simulink model "drone_position_control_ista_tuned"  (R2022a)
settings: Solver=ode4  StartTime=0.0  StopTime=42  FixedStep=.0005  RelTol=1e-3
model workspace (MAT data in the model file):
  AttDyna_Ixx = 0.0211
  AttDyna_Iyy = 0.0219
  AttDyna_Izz = 0.0366
  AttDyna_JRP = 0.0001287
  ConEfficiency_drone_R = 0.225
  ConEfficiency_drone_cM = 1.779e-07
  ConEfficiency_drone_cT = 1.105e-05
  HeightISTAParams = [20 40 0.01 -22 8 8 0.005 3 5]
  HeightNominalPlant = [1.4 9.8 1.105e-05 1148 -141.4]
  HeightSTAParams = [20 12 0.01 -22 8 8 0.005 3 5]
  PosDyna_GravityAcc = 9.8
  PosDyna_Mass = 1.4
  PowerUnit_CR = 1148
  PowerUnit_Tm = 0.02
  PowerUnit_wb = -141.4
  XYISTAParams = [3 1 0.005 -1.7 1.7 1.7 0.005 1.5]
undefined symbols (not defined in the file): earthRadius, Receive, Send
libraries: aerolibfltsims x3, slpidlib x3, aerolibanimutils x1
(part 2 of 2)

== matlab function drone_position_control_ista_tuned/水平和高度控制/ISTA_y_velocity/ISTA_formula ==
  data: e input; u output; nu input; parameters input; nu_next output; velocity input
function [u, nu_next] = ista_velocity_tuned(e, nu, parameters, velocity)
%#codegen
% 改进隐式ISTA：参数 [k1 k2 epsilon amin amax nu_max Ts lambda]。
% epsilon>0 使用边界层隐式解；epsilon=0 为原作者隐式核。
k1=parameters(1);k2=parameters(2);epsilon=parameters(3);
lo=parameters(4);hi=parameters(5);nu_max=parameters(6);
h=parameters(7);lambda=parameters(8);
if epsilon>0
 [u_ista,nu_candidate]=ista_compensated_step(e,nu,k1,k2,h,epsilon);
else
 [u_ista,nu_candidate]=ISTA_author_step(-e,nu,k1,k2,h,0);
end
u_raw=-lambda*velocity+u_ista;
u=min(max(u_raw,lo),hi);
dnu=nu_candidate-nu;
if (u_raw>hi&&dnu>0)||(u_raw<lo&&dnu<0)
 nu_candidate=nu;
end
nu_next=min(max(nu_candidate,-nu_max),nu_max);
end

function [u, nu_candidate, s_pred] = ista_compensated_step(s, nu, k1, k2, Ts, epsilon)
%#codegen
% 工程改进：用积分状态近似补偿未知加速度扰动，修正隐式预测。
% 假设局部误差动力学 s_dot=-u-d；nu在稳态提供-d的补偿。
% 因而采用 d_hat=-nu，预测 s_pred=s-Ts*(u-nu)。
% 与nu_next=nu+Ts*k2*sat(s_pred/epsilon)、u=k1*psi(s_pred)+nu_next联立。
% 把原核输入平移Ts*nu后，消元右端从s-Ts*nu变为s。
% 不读取实际扰动力；nu并不是任何瞬态下都准确的扰动观测器。
% 这是作者名义隐式核的工程扩展，不等同作者原函数。
[u,nu_candidate,s_pred]=ista_regularized_step(s+Ts*nu,nu,k1,k2,Ts,epsilon);
end

function [u, nu_candidate, s_pred] = ista_regularized_step(s, nu, k1, k2, Ts, epsilon)
%#codegen
% 边界层隐式 ISTA 工程扩展；不是作者原函数的原样复制。
% s = 目标速度 - 实际速度，nu 是当前积分状态，Ts 是控制采样周期。
% epsilon > 0 是速度误差边界层宽度，单位与 s 相同。
%
% 将下面三个名义、未限幅的离散方程联合求解：
% s_pred       = s - Ts*u
% nu_candidate = nu + Ts*k2*sat(s_pred/epsilon)
% u            = k1*sqrt(max(abs(s_pred),epsilon))*sat(s_pred/epsilon)
%                + nu_candidate
%
% 外层保留作者 ISTA 的二次根，内层采用线性边界层的精确隐式解。
% epsilon 趋于零时恢复作者名义隐式核；s_pred 不是实际飞机下一步状态。
% 前馈、执行器动态、输出限幅和条件积分由调用者处理；实际饱和闭环
% 不再严格满足以上无约束递推，不能据此宣称无条件有限时间收敛。

assert(Ts > 0 && epsilon > 0);
assert(k1 >= 0 && k2 >= 0);

w = s - Ts*nu;
A = Ts*k1;
B = Ts*Ts*k2;
sqrt_epsilon = sqrt(epsilon);
boundary = epsilon + A*sqrt_epsilon + B;

if abs(w) <= boundary
    % |s_pred| <= epsilon：同时解误差更新与积分更新。
    denominator = 1 + A/sqrt_epsilon + B/epsilon;
    s_pred = w/denominator;
    sigma = s_pred/epsilon;
    psi = s_pred/sqrt_epsilon;
else
    % |s_pred| > epsilon：与作者外层解相同。
    % 有理化避免 sqrt(A^2+4*C)-A 两个相近数相减。
    C = abs(w) - B;
    r = 2*C/(sqrt(A*A + 4*C) + A);
    sigma = sign(w);
    s_pred = sigma*r*r;
    psi = sigma*r;
end

nu_candidate = nu + Ts*k2*sigma;
u = k1*psi + nu_candidate;
end

function [u_k, nu_next, r_k] = ISTA_author_step(x_k, nu_k, lambda_1, lambda_2, h, Delta_k)
% 按作者截图计算 u、nu，调用后执行 x_next = x_k + h*u_k。
% x、nu、u 分别对应此前代码的 x1、x2、f1_step。
% 此处 nu = nu_ctrl + phi 为闭环第二状态，nu_ctrl 才是原 ISTA.m 的积分状态；
% phi 为对象扰动，phi_dot = Delta。截图的 phi(t) 在此对应 Delta(t)。
%
% 输入：x_k, nu_k                 t_k 时刻的闭环状态
%       lambda_1, lambda_2, h     增益及时间步长
%       Delta_k                  扰动导数 Delta(t_k)
% 输出：u_k                      作者截图中的本步增量速率
%       nu_next                  t_{k+1} 时刻的第二状态
%       r_k                      名义隐式步的非负平方根幅值
%
% u_k 一般不等于图 7 的后处理量 u_plot = nu-lambda_1*sqrt(abs(x))*sign(x)，
% 也不直接等同于原对象的物理控制输入。本函数用于复现作者闭环仿真。
% 以下公式及运算顺序保持作者截图的写法。

    a = h * lambda_1;
    b_k = -x_k - h * nu_k;

    if b_k < -h^2 * lambda_2
        r_k = (-a + sqrt(a^2 - 4 * (b_k + lambda_2 * h^2))) / 2;
        nu_next = nu_k - lambda_2 * h + h * Delta_k;
        u_k = -lambda_1 * r_k + nu_next;
    elseif b_k > h^2 * lambda_2
        r_k = (-a + sqrt(a^2 + 4 * (b_k - lambda_2 * h^2))) / 2;
        nu_next = nu_k + lambda_2 * h + h * Delta_k;
        u_k = lambda_1 * r_k + nu_next;
    else
        r_k = 0;
        nu_next = nu_k + b_k / h + h * Delta_k;
        u_k = nu_next;
    end
end

== matlab function drone_position_control_ista_tuned/四旋翼简化模型/姿态动力学/att_dyna ==
  data: Ixx input; Iyy input; Izz input; tao_x input; tao_y input; tao_z input; wbx_dot output; wby_dot output; wbz_dot output
function [wbx_dot,wby_dot,wbz_dot] = att_dyna(Ixx,Iyy,Izz,tao_x,tao_y,tao_z)
% wb = [wbx wby wbz]';
% wb_cha = [   0 -wbz   wby;
%            wbz    0  -wbx;
%           -wby  wbx     0];
% I = [Ixx   0   0;
%        0 Iyy   0;
%        0   0 Izz];
I_inv = [1/Ixx     0     0;
             0 1/Iyy     0;
             0     0 1/Izz];
tao = [tao_x tao_y tao_z]';
% G_x = Jrp * wby * (n1+n2-n3-n4);
% G_y = Jrp * wbx * (-n1-n2+n3+n4);
% G_z = 0;  
% G = [G_x G_y G_z]';
wb_dot = I_inv * (tao);
wbx_dot = wb_dot(1,1);
wby_dot = wb_dot(2,1);
wbz_dot = wb_dot(3,1);
end

== matlab function drone_position_control_ista_tuned/四旋翼简化模型/位置动力学/pos_dyna ==
  data: f input; vx_dot output; m input; g input; yaw input; pitch input; roll input; vy_dot output; vz_dot output
function [vx_dot,vy_dot,vz_dot] = pos_dyna(f,m,g,yaw,pitch,roll)
%位置动力学
%忽略了角速度和线速度的叉乘
vx_dot = (sin(roll)*sin(yaw) + cos(roll)*cos(yaw)*sin(pitch))*f/m;
vy_dot = (cos(roll)*sin(pitch)*sin(yaw) - cos(yaw)*sin(roll))*f/m;
vz_dot = (cos(pitch)*cos(roll)*f/m)+g;
end

== matlab function drone_position_control_ista_tuned/四旋翼简化模型/姿态运动学/att_kine ==
  data: wbx input; roll_dot output; wby input; wbz input; pitch input; pitch_dot output; yaw_dot output; roll input
function [roll_dot,pitch_dot,yaw_dot] = att_kine(wbx,wby,wbz,pitch,roll)
%姿态运动学
roll_dot = wbx + tan(pitch)*sin(roll)*wby + tan(pitch)*cos(roll)*wbz;
pitch_dot = cos(roll)*wby - sin(roll)*wbz;
yaw_dot = (sin(roll)/cos(pitch))*wby + (cos(roll)/cos(pitch))*wbz;
end

== matlab function drone_position_control_ista_tuned/四旋翼简化模型/控制效率模型/control_efficiency ==
  data: n1 input; f output; n2 input; n3 input; n4 input; tao_x output; tao_y output; tao_z output; d input; ct input; cm input
function [f,tao_x,tao_y,tao_z] = control_efficiency(n1,n2,n3,n4,d,ct,cm)
%控制效率模型
%X型机架
%3↓   1↑
%  \ /
%  / \
%2↑   4↓
%转速单位是弧度
f = -1*ct*(n1^2 + n2^2 + n3^2 + n4^2);%z轴朝下，所以拉力为负
tao_x = d*ct*sin(pi/4)*(-n1^2 + n2^2 + n3^2 - n4^2) / 2;
tao_y = d*ct*sin(pi/4)*(n1^2 - n2^2 + n3^2 - n4^2) / 2;
tao_z = cm*(n1^2 + n2^2 - n3^2 - n4^2);
%十字型
% f = ct*(n1^2 + n2^2 + n3^2 + n4^2);
% tao_x = -d*ct*n2^2 + d*ct*n4^2;
% tao_y =  d*ct*n1^2 - d*ct*n3^2;
% tao_z = cm*(n1^2 - n2^2 + n3^2 - n4^2);
end

== matlab function drone_position_control_ista_tuned/动力电机分配 ==
  data: thrust input; m1 output; m2 output; m3 output; m4 output; roll_pwm input; pitch_pwm input; yaw_pwm input
function [m1,m2,m3,m4] = motor_mixer(thrust,roll_pwm,pitch_pwm,yaw_pwm)
%输入的是都是占空比（0-1）之间
%输出四个电机的指令值，1000-2000
%这里采用x型机架，x型机架的分配和十字型的不一样

K = 1000;%将输入定在0-1000
pwm_base = 1000;%PWM从1000开始

m1 = (thrust - roll_pwm + pitch_pwm + yaw_pwm) * K + pwm_base;
m2 = (thrust + roll_pwm - pitch_pwm + yaw_pwm) * K + pwm_base;
m3 = (thrust + roll_pwm + pitch_pwm - yaw_pwm) * K + pwm_base;
m4 = (thrust - roll_pwm - pitch_pwm - yaw_pwm) * K + pwm_base;
end

== matlab function drone_position_control_ista_tuned/水平和高度控制/MATLAB Function ==
  data: v_x input; roll_d output; v_y input; act_yaw input; g input; pitch_d output
function [roll_d, pitch_d] = fcn(v_x,v_y,act_yaw,g)
%v_x,v_y是经过速度环pid控制之后的输出
%yaw是实际的yaw角度,单位是弧度制,并且matlab的三角函数接收的是弧度制
%g是重力加速度
%输出的角度也是弧度制
A_INV = [sin(act_yaw) -cos(act_yaw);
         cos(act_yaw)  sin(act_yaw)];
desire_roll_pitch = -1*(1/g) * A_INV * [v_x;v_y]; 
roll_d = desire_roll_pitch(1);
pitch_d = desire_roll_pitch(2);
